simulink model "StarshipSystemModel"  (R2025b)
settings: Solver=VariableStepAuto  StartTime=0.0  StopTime=10.0  RelTol=1e-3
model workspace (MAT data in the model file):
  ActiveGNCMode : Simulink.Bus (value not decoded)
  AerodynamicControlCommand : Simulink.Bus (value not decoded)
  AerodynamicLoad : Simulink.Bus (value not decoded)
  AggregatedStream : Simulink.Bus (value not decoded)
  AllocatedEffectorDemand : Simulink.Bus (value not decoded)
  AttitudeControlDemand : Simulink.Bus (value not decoded)
  AttitudeGuidanceCommand : Simulink.Bus (value not decoded)
  AttitudeRateState : Simulink.Bus (value not decoded)
  AutogenousPressurantGas : Simulink.ConnectionBus (value not decoded)
  CandidateFaultIndication : Simulink.Bus (value not decoded)
  CombustionGasFeed : Simulink.ConnectionBus (value not decoded)
  CommandPathHealth : Simulink.Bus (value not decoded)
  ControlMode : Simulink.ValueType (value not decoded)
  DownlinkSignal : Simulink.Bus (value not decoded)
  ElectricalPower : Simulink.ConnectionBus (value not decoded)
  EngineTelemetry : Simulink.Bus (value not decoded)
  ExecutionContext : Simulink.Bus (value not decoded)
  FaultDiagnosisResult : Simulink.Bus (value not decoded)
  GNCDataContext : Simulink.Bus (value not decoded)
  GNCHealthState : Simulink.Bus (value not decoded)
  GNCStateEstimate : Simulink.Bus (value not decoded)
  GimbalAngle : Simulink.ValueType (value not decoded)
  GimbalMotion : Simulink.ConnectionBus (value not decoded)
  GroundCheckoutLink : Simulink.Bus (value not decoded)
  GroundPressurantSupply : Simulink.ConnectionBus (value not decoded)
  GuidanceConstraints : Simulink.Bus (value not decoded)
  GuidanceMode : Simulink.ValueType (value not decoded)
  LinkHealth : Simulink.Bus (value not decoded)
  LiquidPropellantFeed : Simulink.ConnectionBus (value not decoded)
  MechanicalMotion : Simulink.ConnectionBus (value not decoded)
  MechanismPosition : Simulink.Bus (value not decoded)
  ModeTransitionContext : Simulink.Bus (value not decoded)
  NavigationAidingData : Simulink.Bus (value not decoded)
  NavigationEstimate : Simulink.Bus (value not decoded)
  NavigationHealthStatus : Simulink.Bus (value not decoded)
  NavigationMeasurementSet : Simulink.Bus (value not decoded)
  PercentThrottle : Simulink.ValueType (value not decoded)
  PneumaticActuationGas : Simulink.ConnectionBus (value not decoded)
  PowerConversionStatus : Simulink.Bus (value not decoded)
  PowerDistributionStatus : Simulink.Bus (value not decoded)
  PowerHealthStatus : Simulink.Bus (value not decoded)
  PowerManagementCommand : Simulink.Bus (value not decoded)
  PowerStorageStatus : Simulink.Bus (value not decoded)
  ProtectedThermalState : Simulink.Bus (value not decoded)
  ProtectionIsolationStatus : Simulink.Bus (value not decoded)
  PurgeGasSupply : Simulink.ConnectionBus (value not decoded)
  RCSPulseCommand : Simulink.Bus (value not decoded)
  RCSTelemetry : Simulink.Bus (value not decoded)
  RFFeed : Simulink.ConnectionBus (value not decoded)
  RecoveryMechanismCommand : Simulink.Bus (value not decoded)
  RollThrottleBias : Simulink.ValueType (value not decoded)
  SafetyOverride : Simulink.ValueType (value not decoded)
  SafetyStateStatus : Simulink.Bus (value not decoded)
  ShapedControlDemand : Simulink.Bus (value not decoded)
  SpinStartIgniterGas : Simulink.ConnectionBus (value not decoded)
  StageMechanicalBoundary : Simulink.ConnectionBus (value not decoded)
  StructuralLoad : Simulink.ConnectionBus (value not decoded)
  StructureHealthStatus : Simulink.Bus (value not decoded)
  SubsystemHealthEvidence : Simulink.Bus (value not decoded)
  SubsystemStatusTelemetry : Simulink.Bus (value not decoded)
  TankTelemetry : Simulink.Bus (value not decoded)
  ThermalMonitoringCommand : Simulink.Bus (value not decoded)
  ThermalNetwork : Simulink.ConnectionBus (value not decoded)
  ThrustLoad : Simulink.ConnectionBus (value not decoded)
  TrajectoryGuidanceCommand : Simulink.Bus (value not decoded)
  TrajectoryReference : Simulink.Bus (value not decoded)
  TranslationalControlDemand : Simulink.Bus (value not decoded)
  TranslationalState : Simulink.Bus (value not decoded)
  UplinkSignal : Simulink.Bus (value not decoded)
  ValidatedControlDemand : Simulink.Bus (value not decoded)
  ValveCommand : Simulink.ValueType (value not decoded)
  VehicleStructureState : Simulink.Bus (value not decoded)
  VerifiedCommand : Simulink.Bus (value not decoded)
  VideoStream : Simulink.Bus (value not decoded)
undefined symbols (not defined in the file): ACR, ACT, ASM, ATM, BCR, BDQ, BDR, BDX, BEC, BFC, BHV, BIP, BLM, BNZ, BPI, BPR, BPV, BRX, BSM, BTA, BTP, BVC, BVE, BVV, CAA, CAM, CAS, CAT, CLM, COM, CRS, CTL, CTR, DAQ, ESC, EXT, FCR, FDB, FDE, FEX, FHI, FHM, FIC, FIS, FMG, FSC, GAP, GCM, GMD, GNC, GND, GPH, GTR, HDN, HIA, HSI, IF, INT, LOC, NAI ... (+45)
(part 7 of 8)

== system StarshipSystemModel/Starship/Power & Electrical Energy/Power Conversion & Conditioning/Inverter // Conversion Function ==
  IF-BES-INV-01 : PMIOPort  Side=Left  ConnectionType=Bus: ElectricalPower
  IF-INV-PCR-01 : PMIOPort  Port=2  Side=Right  ConnectionType=Bus: ElectricalPower

== system StarshipSystemModel/Starship/Power & Electrical Energy/Power Conversion & Conditioning/Power Conditioning // Regulation ==
  IF-INV-PCR-01 : PMIOPort  Side=Left  ConnectionType=Bus: ElectricalPower
  IF-PCR-HDN-01 : PMIOPort  Port=2  Side=Right  ConnectionType=Bus: ElectricalPower

== system StarshipSystemModel/Starship/Power & Electrical Energy/Power Management & Monitoring/Power Management Coordinator ==
  Bus Element In1 : Inport  PortName=IF-PSM-PMC-01
  Bus Element Out1 : Outport  PortName=IF-PMC-BIP-01
  Bus Element Out2 : Outport  Port=2  PortName=IF-PMC-HSI-01
  Bus Element Out3 : Outport  Port=3  PortName=IF-PMM-SAF-01

== system StarshipSystemModel/Starship/Power & Electrical Energy/Power Management & Monitoring/Power State Monitor ==
  Bus Element In3 : Inport  PortName=IF-HDN-PSM-01
  Bus Element In2 : Inport  Port=2  PortName=IF-PCM-PSM-01
  Bus Element In1 : Inport  Port=3  PortName=IF-BSM-PSM-01
  Bus Element Out1 : Outport  PortName=IF-PSM-PMC-01

== system StarshipSystemModel/Starship/Power & Electrical Energy/Power Management & Monitoring/Protection // Isolation Status ==
  Bus Element In1 : Inport  PortName=IF-BIP-PIS-01
  Bus Element In2 : Inport  Port=2  PortName=IF-HSI-PIS-01
  Bus Element In3 : Inport  Port=3  PortName=IF-BPI-PIS-01

== system StarshipSystemModel/Starship/Propellent system/Booster propellant System/Booster propellant tanks ==
  Anti-slosh baffles : Subsystem
      settings: PortSchema="{\"entries\":[{\"content\":{\"headerSize\":26,\"margin\":15,\"minimumSpacing\":25,\"sides\":[{\"content\":{},\"type\":\"ConnectorPlacement.EquallySpacedRectSide\",\"uuid\":\"fbe4f8e6-132c-4a0c-8c4c-52d0209da778\"},{\"content\":{\"side\":\"RIGHT\"},\"type\":\"ConnectorPlacement.EquallySpacedRectSide\",\"uuid\":\"bbe80fa3-b8e3-44c5-9574-5758a55378fd\"},{\"content\":{\"side\":\"TOP\"},\"type\":\"ConnectorPlacement.EquallySpacedRectSide\",\"uuid\":\"410005e2-e10b-4d3e-a617-d51b1ea5de7e\"}]},\"type\":\"ConnectorPlacement.EquallySpacedConnector\",\"uuid\":\"b66a347a-e5b4-46b1-8a3f-28cf70f30a27\"}],\"packageUris\":[\"http://schema.mathworks.com/mf0/Connector/R2020b\"],\"version\":\"1.0\"}"
  CH4 main tank : Subsystem
      settings: PortSchema="{\"entries\":[{\"content\":{\"headerSize\":26,\"margin\":15,\"minimumSpacing\":25,\"sides\":[{\"content\":{\"connectorIds\":[\"LConn1\",\"LConn2\"]},\"type\":\"ConnectorPlacement.EquallySpacedRectSide\",\"uuid\":\"fbe4f8e6-132c-4a0c-8c4c-52d0209da778\"},{\"content\":{\"connectorIds\":[\"RConn1\",\"RConn2\"],\"side\":\"RIGHT\"},\"type\":\"ConnectorPlacement.EquallySpacedRectSide\",\"uuid\":\"bbe80fa3-b8e3-44c5-9574-5758a55378fd\"},{\"content\":{\"side\":\"TOP\"},\"type\":\"ConnectorPlacement.EquallySpacedRectSide\",\"uuid\":\"410005e2-e10b-4d3e-a617-d51b1ea5de7e\"}]},\"type\":\"ConnectorPlacement.EquallySpacedConnector\",\"uuid\":\"b66a347a-e5b4-46b1-8a3f-28cf70f30a27\"}],\"packageUris\":[\"http://schema.mathworks.com/mf0/Connector/R2020b\"],\"version\":\"1.0\"}"
  CH4 transfer tube (downcomer) : Subsystem
      settings: PortSchema="{\"entries\":[{\"content\":{\"headerSize\":26,\"margin\":15,\"minimumSpacing\":25,\"sides\":[{\"content\":{},\"type\":\"ConnectorPlacement.EquallySpacedRectSide\",\"uuid\":\"fbe4f8e6-132c-4a0c-8c4c-52d0209da778\"},{\"content\":{\"side\":\"RIGHT\"},\"type\":\"ConnectorPlacement.EquallySpacedRectSide\",\"uuid\":\"bbe80fa3-b8e3-44c5-9574-5758a55378fd\"},{\"content\":{\"side\":\"TOP\"},\"type\":\"ConnectorPlacement.EquallySpacedRectSide\",\"uuid\":\"410005e2-e10b-4d3e-a617-d51b1ea5de7e\"}]},\"type\":\"ConnectorPlacement.EquallySpacedConnector\",\"uuid\":\"b66a347a-e5b4-46b1-8a3f-28cf70f30a27\"}],\"packageUris\":[\"http://schema.mathworks.com/mf0/Connector/R2020b\"],\"version\":\"1.0\"}"
  Common dome : Subsystem
      settings: PortSchema="{\"entries\":[{\"content\":{\"headerSize\":26,\"margin\":15,\"minimumSpacing\":25,\"sides\":[{\"content\":{},\"type\":\"ConnectorPlacement.EquallySpacedRectSide\",\"uuid\":\"fbe4f8e6-132c-4a0c-8c4c-52d0209da778\"},{\"content\":{\"side\":\"RIGHT\"},\"type\":\"ConnectorPlacement.EquallySpacedRectSide\",\"uuid\":\"bbe80fa3-b8e3-44c5-9574-5758a55378fd\"},{\"content\":{\"side\":\"TOP\"},\"type\":\"ConnectorPlacement.EquallySpacedRectSide\",\"uuid\":\"410005e2-e10b-4d3e-a617-d51b1ea5de7e\"}]},\"type\":\"ConnectorPlacement.EquallySpacedConnector\",\"uuid\":\"b66a347a-e5b4-46b1-8a3f-28cf70f30a27\"}],\"packageUris\":[\"http://schema.mathworks.com/mf0/Connector/R2020b\"],\"version\":\"1.0\"}"
  LOX landing tank : Subsystem
      settings: PortSchema="{\"entries\":[{\"content\":{\"headerSize\":26,\"margin\":15,\"minimumSpacing\":25,\"sides\":[{\"content\":{},\"type\":\"ConnectorPlacement.EquallySpacedRectSide\",\"uuid\":\"fbe4f8e6-132c-4a0c-8c4c-52d0209da778\"},{\"content\":{\"connectorIds\":[\"RConn1\"],\"side\":\"RIGHT\"},\"type\":\"ConnectorPlacement.EquallySpacedRectSide\",\"uuid\":\"bbe80fa3-b8e3-44c5-9574-5758a55378fd\"},{\"content\":{\"side\":\"TOP\"},\"type\":\"ConnectorPlacement.EquallySpacedRectSide\",\"uuid\":\"410005e2-e10b-4d3e-a617-d51b1ea5de7e\"}]},\"type\":\"ConnectorPlacement.EquallySpacedConnector\",\"uuid\":\"b66a347a-e5b4-46b1-8a3f-28cf70f30a27\"}],\"packageUris\":[\"http://schema.mathworks.com/mf0/Connector/R2020b\"],\"version\":\"1.0\"}"
  LOX main tank : Subsystem
      settings: PortSchema="{\"entries\":[{\"content\":{\"headerSize\":26,\"margin\":15,\"minimumSpacing\":25,\"sides\":[{\"content\":{\"connectorIds\":[\"LConn2\",\"LConn3\"]},\"type\":\"ConnectorPlacement.EquallySpacedRectSide\",\"uuid\":\"fbe4f8e6-132c-4a0c-8c4c-52d0209da778\"},{\"content\":{\"connectorIds\":[\"LConn1\",\"RConn1\",\"RConn2\"],\"side\":\"RIGHT\"},\"type\":\"ConnectorPlacement.EquallySpacedRectSide\",\"uuid\":\"bbe80fa3-b8e3-44c5-9574-5758a55378fd\"},{\"content\":{\"side\":\"TOP\"},\"type\":\"ConnectorPlacement.EquallySpacedRectSide\",\"uuid\":\"410005e2-e10b-4d3e-a617-d51b1ea5de7e\"}]},\"type\":\"ConnectorPlacement.EquallySpacedConnector\",\"uuid\":\"b66a347a-e5b4-46b1-8a3f-28cf70f30a27\"}],\"packageUris\":[\"http://schema.mathworks.com/mf0/Connector/R2020b\"],\"version\":\"1.0\"}"
  IF-BOT-BPV-01 : PMIOPort  Side=Right
  IF-BFT-BPV-01 : PMIOPort  Port=2  Side=Right  ConnectionType=Bus: LiquidPropellantFeed
  IF-BFT-BVV-01 : PMIOPort  Port=3  Side=Right  ConnectionType=Bus: AutogenousPressurantGas
  IF-BOT-BVV-01 : PMIOPort  Port=4  Side=Right  ConnectionType=Bus: AutogenousPressurantGas
  IF-BLT-BHV-01 : PMIOPort  Port=5  Side=Right  ConnectionType=Bus: LiquidPropellantFeed
  IF-BOT-PRS-01 : PMIOPort  Port=6  Side=Left  ConnectionType=Bus: StructuralLoad
  IF-BCQ-BFT-01 : PMIOPort  Port=7  Side=Left  ConnectionType=Bus: LiquidPropellantFeed
  IF-BPR-BOT-01 : PMIOPort  Port=8  Side=Left  ConnectionType=Bus: AutogenousPressurantGas
  IF-BLQ-BOT-01 : PMIOPort  Port=9  Side=Left  ConnectionType=Bus: LiquidPropellantFeed
  IF-BPR-BFT-01 : PMIOPort  Port=10  Side=Left  ConnectionType=Bus: AutogenousPressurantGas
  connections:
  IF-BPR-BOT-01/RConn1 -- LOX main tank/LConn2
  IF-BPR-BFT-01/RConn1 -- CH4 main tank/LConn2
  IF-BLQ-BOT-01/RConn1 -- LOX main tank/LConn3
  IF-BCQ-BFT-01/RConn1 -- CH4 main tank/LConn1
  CH4 main tank/RConn1 -- IF-BFT-BPV-01/RConn1
  LOX landing tank/RConn1 -- IF-BLT-BHV-01/RConn1
  LOX main tank/RConn1 -- IF-BOT-BPV-01/RConn1
  LOX main tank/RConn2 -- IF-BOT-BVV-01/RConn1
  CH4 main tank/RConn2 -- IF-BFT-BVV-01/RConn1
  IF-BOT-PRS-01/RConn1 -- LOX main tank/LConn1

== system StarshipSystemModel/Starship/Propellent system/Booster propellant System/Feed & distribution ==
  Bus Element In1 : Inport  PortName=IF-GNC-BFC-01
  Distribution manifold : Subsystem
      settings: PortSchema="{\"entries\":[{\"content\":{\"headerSize\":26,\"margin\":15,\"minimumSpacing\":25,\"sides\":[{\"content\":{\"connectorIds\":[\"LConn1\",\"LConn2\"]},\"type\":\"ConnectorPlacement.EquallySpacedRectSide\",\"uuid\":\"fbe4f8e6-132c-4a0c-8c4c-52d0209da778\"},{\"content\":{\"connectorIds\":[\"RConn1\"],\"side\":\"RIGHT\"},\"type\":\"ConnectorPlacement.EquallySpacedRectSide\",\"uuid\":\"bbe80fa3-b8e3-44c5-9574-5758a55378fd\"},{\"content\":{\"side\":\"TOP\"},\"type\":\"ConnectorPlacement.EquallySpacedRectSide\",\"uuid\":\"410005e2-e10b-4d3e-a617-d51b1ea5de7e\"}]},\"type\":\"ConnectorPlacement.EquallySpacedConnector\",\"uuid\":\"b66a347a-e5b4-46b1-8a3f-28cf70f30a27\"}],\"packageUris\":[\"http://schema.mathworks.com/mf0/Connector/R2020b\"],\"version\":\"1.0\"}"
  Feed controller : Subsystem
      settings: PortSchema="{\"entries\":[{\"content\":{\"headerSize\":26,\"margin\":15,\"minimumSpacing\":25,\"sides\":[{\"content\":{\"connectorIds\":[\"In1\",\"LConn1\"]},\"type\":\"ConnectorPlacement.EquallySpacedRectSide\",\"uuid\":\"fbe4f8e6-132c-4a0c-8c4c-52d0209da778\"},{\"content\":{\"connectorIds\":[\"Out1\",\"Out2\"],\"side\":\"RIGHT\"},\"type\":\"ConnectorPlacement.EquallySpacedRectSide\",\"uuid\":\"bbe80fa3-b8e3-44c5-9574-5758a55378fd\"},{\"content\":{\"side\":\"TOP\"},\"type\":\"ConnectorPlacement.EquallySpacedRectSide\",\"uuid\":\"410005e2-e10b-4d3e-a617-d51b1ea5de7e\"}]},\"type\":\"ConnectorPlacement.EquallySpacedConnector\",\"uuid\":\"b66a347a-e5b4-46b1-8a3f-28cf70f30a27\"}],\"packageUris\":[\"http://schema.mathworks.com/mf0/Connector/R2020b\"],\"version\":\"1.0\"}"
  Header tank switchover valve : Subsystem
      settings: PortSchema="{\"entries\":[{\"content\":{\"headerSize\":26,\"margin\":15,\"minimumSpacing\":25,\"sides\":[{\"content\":{\"connectorIds\":[\"LConn1\",\"In1\",\"LConn2\"]},\"type\":\"ConnectorPlacement.EquallySpacedRectSide\",\"uuid\":\"fbe4f8e6-132c-4a0c-8c4c-52d0209da778\"},{\"content\":{\"connectorIds\":[\"RConn1\"],\"side\":\"RIGHT\"},\"type\":\"ConnectorPlacement.EquallySpacedRectSide\",\"uuid\":\"bbe80fa3-b8e3-44c5-9574-5758a55378fd\"},{\"content\":{\"side\":\"TOP\"},\"type\":\"ConnectorPlacement.EquallySpacedRectSide\",\"uuid\":\"410005e2-e10b-4d3e-a617-d51b1ea5de7e\"}]},\"type\":\"ConnectorPlacement.EquallySpacedConnector\",\"uuid\":\"b66a347a-e5b4-46b1-8a3f-28cf70f30a27\"}],\"packageUris\":[\"http://schema.mathworks.com/mf0/Connector/R2020b\"],\"version\":\"1.0\"}"
  Main tank outlet valve (prevalve) : Subsystem
      settings: PortSchema="{\"entries\":[{\"content\":{\"headerSize\":26,\"margin\":15,\"minimumSpacing\":25,\"sides\":[{\"content\":{\"connectorIds\":[\"LConn1\",\"LConn2\",\"In1\",\"LConn3\"]},\"type\":\"ConnectorPlacement.EquallySpacedRectSide\",\"uuid\":\"fbe4f8e6-132c-4a0c-8c4c-52d0209da778\"},{\"content\":{\"connectorIds\":[\"RConn1\"],\"side\":\"RIGHT\"},\"type\":\"ConnectorPlacement.EquallySpacedRectSide\",\"uuid\":\"bbe80fa3-b8e3-44c5-9574-5758a55378fd\"},{\"content\":{\"side\":\"TOP\"},\"type\":\"ConnectorPlacement.EquallySpacedRectSide\",\"uuid\":\"410005e2-e10b-4d3e-a617-d51b1ea5de7e\"}]},\"type\":\"ConnectorPlacement.EquallySpacedConnector\",\"uuid\":\"b66a347a-e5b4-46b1-8a3f-28cf70f30a27\"}],\"packageUris\":[\"http://schema.mathworks.com/mf0/Connector/R2020b\"],\"version\":\"1.0\"}"
  IF-BDM-BTP-01 : PMIOPort  Side=Right  ConnectionType=Bus: LiquidPropellantFeed
  IF-BOT-BPV-01 : PMIOPort  Port=2  Side=Left  ConnectionType=Bus: LiquidPropellantFeed
  IF-BLT-BHV-01 : PMIOPort  Port=3  Side=Left  ConnectionType=Bus: LiquidPropellantFeed
  IF-BNG-BPV-01 : PMIOPort  Port=4  Side=Left  ConnectionType=Bus: PneumaticActuationGas
  IF-BNG-BHV-01 : PMIOPort  Port=5  Side=Left  ConnectionType=Bus: PneumaticActuationGas
  IF-BFT-BPV-01 : PMIOPort  Port=6  Side=Left  ConnectionType=Bus: LiquidPropellantFeed
  IF-PWR-BFC-01 : PMIOPort  Port=7  Side=Left  ConnectionType=Bus: ElectricalPower
  wires:
  Bus Element In1/1 -> Feed controller/1(IF-GNC-BFC-01)
  Feed controller/2(IF-BFC-BHV-01) -> Header tank switchover valve/1(IF-BFC-BHV-01)
  Feed controller/1(IF-BFC-BPV-01) -> Main tank outlet valve (prevalve)/1(IF-BFC-BPV-01)
  connections:
  IF-BLT-BHV-01/RConn1 -- Header tank switchover valve/LConn1
  IF-BFT-BPV-01/RConn1 -- Main tank outlet valve (prevalve)/LConn2
  Header tank switchover valve/RConn1 -- Distribution manifold/LConn1
  IF-BNG-BHV-01/RConn1 -- Header tank switchover valve/LConn2
  IF-BOT-BPV-01/RConn1 -- Main tank outlet valve (prevalve)/LConn1
  IF-BNG-BPV-01/RConn1 -- Main tank outlet valve (prevalve)/LConn3
  Main tank outlet valve (prevalve)/RConn1 -- Distribution manifold/LConn2
  Distribution manifold/RConn1 -- IF-BDM-BTP-01/RConn1
  IF-PWR-BFC-01/RConn1 -- Feed controller/LConn1

== system StarshipSystemModel/Starship/Propellent system/Booster propellant System/Ground propellant interface ==
  CH4 quick-disconnect panel : Subsystem
      settings: PortSchema="{\"entries\":[{\"content\":{\"headerSize\":26,\"margin\":15,\"minimumSpacing\":25,\"sides\":[{\"content\":{\"connectorIds\":[\"LConn1\"]},\"type\":\"ConnectorPlacement.EquallySpacedRectSide\",\"uuid\":\"fbe4f8e6-132c-4a0c-8c4c-52d0209da778\"},{\"content\":{\"connectorIds\":[\"RConn1\"],\"side\":\"RIGHT\"},\"type\":\"ConnectorPlacement.EquallySpacedRectSide\",\"uuid\":\"bbe80fa3-b8e3-44c5-9574-5758a55378fd\"},{\"content\":{\"side\":\"TOP\"},\"type\":\"ConnectorPlacement.EquallySpacedRectSide\",\"uuid\":\"410005e2-e10b-4d3e-a617-d51b1ea5de7e\"}]},\"type\":\"ConnectorPlacement.EquallySpacedConnector\",\"uuid\":\"b66a347a-e5b4-46b1-8a3f-28cf70f30a27\"}],\"packageUris\":[\"http://schema.mathworks.com/mf0/Connector/R2020b\"],\"version\":\"1.0\"}"
  LOX quick-disconnect panel : Subsystem
      settings: PortSchema="{\"entries\":[{\"content\":{\"headerSize\":26,\"margin\":15,\"minimumSpacing\":25,\"sides\":[{\"content\":{\"connectorIds\":[\"LConn1\"]},\"type\":\"ConnectorPlacement.EquallySpacedRectSide\",\"uuid\":\"fbe4f8e6-132c-4a0c-8c4c-52d0209da778\"},{\"content\":{\"connectorIds\":[\"RConn1\"],\"side\":\"RIGHT\"},\"type\":\"ConnectorPlacement.EquallySpacedRectSide\",\"uuid\":\"bbe80fa3-b8e3-44c5-9574-5758a55378fd\"},{\"content\":{\"side\":\"TOP\"},\"type\":\"ConnectorPlacement.EquallySpacedRectSide\",\"uuid\":\"410005e2-e10b-4d3e-a617-d51b1ea5de7e\"}]},\"type\":\"ConnectorPlacement.EquallySpacedConnector\",\"uuid\":\"b66a347a-e5b4-46b1-8a3f-28cf70f30a27\"}],\"packageUris\":[\"http://schema.mathworks.com/mf0/Connector/R2020b\"],\"version\":\"1.0\"}"
  Purge/pressurant ground QD : Subsystem
      settings: PortSchema="{\"entries\":[{\"content\":{\"headerSize\":26,\"margin\":15,\"minimumSpacing\":25,\"sides\":[{\"content\":{\"connectorIds\":[\"LConn1\"]},\"type\":\"ConnectorPlacement.EquallySpacedRectSide\",\"uuid\":\"fbe4f8e6-132c-4a0c-8c4c-52d0209da778\"},{\"content\":{\"connectorIds\":[\"RConn1\",\"RConn2\",\"RConn3\"],\"side\":\"RIGHT\"},\"type\":\"ConnectorPlacement.EquallySpacedRectSide\",\"uuid\":\"bbe80fa3-b8e3-44c5-9574-5758a55378fd\"},{\"content\":{\"side\":\"TOP\"},\"type\":\"ConnectorPlacement.EquallySpacedRectSide\",\"uuid\":\"410005e2-e10b-4d3e-a617-d51b1ea5de7e\"}]},\"type\":\"ConnectorPlacement.EquallySpacedConnector\",\"uuid\":\"b66a347a-e5b4-46b1-8a3f-28cf70f30a27\"}],\"packageUris\":[\"http://schema.mathworks.com/mf0/Connector/R2020b\"],\"version\":\"1.0\"}"
  "IF-GND-BLQ-01\t" : PMIOPort  Side=Left
  "IF-GND-BCQ-01\t" : PMIOPort  Port=2  Side=Left
  IF-GND-BPQ-01 : PMIOPort  Port=3  Side=Left  ConnectionType=Bus: GroundPressurantSupply
  IF-BCQ-BFT-01 : PMIOPort  Port=4  Side=Right  ConnectionType=Bus: LiquidPropellantFeed
  IF-BPQ-BSG-01 : PMIOPort  Port=5  Side=Right  ConnectionType=Bus: GroundPressurantSupply
  IF-BPQ-BNG-01 : PMIOPort  Port=6  Side=Right  ConnectionType=Bus: GroundPressurantSupply
  IF-BPQ-BPR-01 : PMIOPort  Port=7  Side=Right  ConnectionType=Bus: GroundPressurantSupply
  IF-BLQ-BOT-01 : PMIOPort  Port=8  Side=Right  ConnectionType=Bus: LiquidPropellantFeed
  connections:
  Purge/pressurant ground QD/RConn1 -- IF-BPQ-BSG-01/RConn1
  IF-GND-BPQ-01/RConn1 -- Purge/pressurant ground QD/LConn1
  "IF-GND-BLQ-01\t"/RConn1 -- LOX quick-disconnect panel/LConn1
  Purge/pressurant ground QD/RConn3 -- IF-BPQ-BNG-01/RConn1
  CH4 quick-disconnect panel/RConn1 -- IF-BCQ-BFT-01/RConn1
  "IF-GND-BCQ-01\t"/RConn1 -- CH4 quick-disconnect panel/LConn1
  Purge/pressurant ground QD/RConn2 -- IF-BPQ-BPR-01/RConn1
  LOX quick-disconnect panel/RConn1 -- IF-BLQ-BOT-01/RConn1

== system StarshipSystemModel/Starship/Propellent system/Booster propellant System/Pressurization, purge & venting ==
  Bus Element In1 : Inport  PortName=IF-GNC-BPR-01
  Autogenous pressurization regulator : Subsystem
      settings: PortSchema="{\"entries\":[{\"content\":{\"headerSize\":26,\"margin\":15,\"minimumSpacing\":25,\"sides\":[{\"content\":{\"connectorIds\":[\"LConn1\",\"LConn2\",\"In1\",\"LConn3\"]},\"type\":\"ConnectorPlacement.EquallySpacedRectSide\",\"uuid\":\"fbe4f8e6-132c-4a0c-8c4c-52d0209da778\"},{\"content\":{\"connectorIds\":[\"Out1\",\"Out2\",\"RConn1\",\"RConn2\",\"Out3\"],\"side\":\"RIGHT\"},\"type\":\"ConnectorPlacement.EquallySpacedRectSide\",\"uuid\":\"bbe80fa3-b8e3-44c5-9574-5758a55378fd\"},{\"content\":{\"side\":\"TOP\"},\"type\":\"ConnectorPlacement.EquallySpacedRectSide\",\"uuid\":\"410005e2-e10b-4d3e-a617-d51b1ea5de7e\"}]},\"type\":\"ConnectorPlacement.EquallySpacedConnector\",\"uuid\":\"b66a347a-e5b4-46b1-8a3f-28cf70f30a27\"}],\"packageUris\":[\"http://schema.mathworks.com/mf0/Connector/R2020b\"],\"version\":\"1.0\"}"
  Pneumatic actuation gas COPVs : Subsystem
      settings: PortSchema="{\"entries\":[{\"content\":{\"headerSize\":26,\"margin\":15,\"minimumSpacing\":25,\"sides\":[{\"content\":{\"connectorIds\":[\"LConn1\"]},\"type\":\"ConnectorPlacement.EquallySpacedRectSide\",\"uuid\":\"fbe4f8e6-132c-4a0c-8c4c-52d0209da778\"},{\"content\":{\"connectorIds\":[\"RConn1\",\"RConn2\",\"RConn3\",\"RConn4\"],\"side\":\"RIGHT\"},\"type\":\"ConnectorPlacement.EquallySpacedRectSide\",\"uuid\":\"bbe80fa3-b8e3-44c5-9574-5758a55378fd\"},{\"content\":{\"side\":\"TOP\"},\"type\":\"ConnectorPlacement.EquallySpacedRectSide\",\"uuid\":\"410005e2-e10b-4d3e-a617-d51b1ea5de7e\"}]},\"type\":\"ConnectorPlacement.EquallySpacedConnector\",\"uuid\":\"b66a347a-e5b4-46b1-8a3f-28cf70f30a27\"}],\"packageUris\":[\"http://schema.mathworks.com/mf0/Connector/R2020b\"],\"version\":\"1.0\"}"
  Spin-start & igniter gas COPVs : Subsystem
      settings: PortSchema="{\"entries\":[{\"content\":{\"headerSize\":26,\"margin\":15,\"minimumSpacing\":25,\"sides\":[{\"content\":{\"connectorIds\":[\"LConn1\"]},\"type\":\"ConnectorPlacement.EquallySpacedRectSide\",\"uuid\":\"fbe4f8e6-132c-4a0c-8c4c-52d0209da778\"},{\"content\":{\"connectorIds\":[\"RConn1\"],\"side\":\"RIGHT\"},\"type\":\"ConnectorPlacement.EquallySpacedRectSide\",\"uuid\":\"bbe80fa3-b8e3-44c5-9574-5758a55378fd\"},{\"content\":{\"side\":\"TOP\"},\"type\":\"ConnectorPlacement.EquallySpacedRectSide\",\"uuid\":\"410005e2-e10b-4d3e-a617-d51b1ea5de7e\"}]},\"type\":\"ConnectorPlacement.EquallySpacedConnector\",\"uuid\":\"b66a347a-e5b4-46b1-8a3f-28cf70f30a27\"}],\"packageUris\":[\"http://schema.mathworks.com/mf0/Connector/R2020b\"],\"version\":\"1.0\"}"
  Vent & relief valves : Subsystem
      settings: PortSchema="{\"entries\":[{\"content\":{\"headerSize\":26,\"margin\":15,\"minimumSpacing\":25,\"sides\":[{\"content\":{\"connectorIds\":[\"In1\",\"LConn1\",\"LConn2\",\"LConn3\"]},\"type\":\"ConnectorPlacement.EquallySpacedRectSide\",\"uuid\":\"fbe4f8e6-132c-4a0c-8c4c-52d0209da778\"},{\"content\":{\"side\":\"RIGHT\"},\"type\":\"ConnectorPlacement.EquallySpacedRectSide\",\"uuid\":\"bbe80fa3-b8e3-44c5-9574-5758a55378fd\"},{\"content\":{\"side\":\"TOP\"},\"type\":\"ConnectorPlacement.EquallySpacedRectSide\",\"uuid\":\"410005e2-e10b-4d3e-a617-d51b1ea5de7e\"}]},\"type\":\"ConnectorPlacement.EquallySpacedConnector\",\"uuid\":\"b66a347a-e5b4-46b1-8a3f-28cf70f30a27\"}],\"packageUris\":[\"http://schema.mathworks.com/mf0/Connector/R2020b\"],\"version\":\"1.0\"}"
  IF-BSG-BIG-01 : PMIOPort  Side=Right  ConnectionType=Bus: SpinStartIgniterGas
  IF-BPR-BFT-01 : PMIOPort  Port=2  Side=Right  ConnectionType=Bus: AutogenousPressurantGas
  IF-BNG-BPV-01 : PMIOPort  Port=3  Side=Right  ConnectionType=Bus: PneumaticActuationGas
  IF-BNG-BHV-01 : PMIOPort  Port=4  Side=Right  ConnectionType=Bus: PneumaticActuationGas
  IF-BPR-BOT-01 : PMIOPort  Port=5  Side=Right  ConnectionType=Bus: AutogenousPressurantGas
  IF-BNG-BVC-01 : PMIOPort  Port=6  Side=Right  ConnectionType=Bus: PneumaticActuationGas
  IF-BPQ-BPR-01 : PMIOPort  Port=7  Side=Left  ConnectionType=Bus: GroundPressurantSupply
  IF-BPQ-BNG-01 : PMIOPort  Port=8  Side=Left  ConnectionType=Bus: GroundPressurantSupply
  IF-BPQ-BSG-01 : PMIOPort  Port=9  Side=Left  ConnectionType=Bus: GroundPressurantSupply
  IF-BTP-BPR-01 : PMIOPort  Port=10  Side=Left  ConnectionType=Bus: AutogenousPressurantGas
  IF-BOT-BVV-01 : PMIOPort  Port=11  Side=Left  ConnectionType=Bus: AutogenousPressurantGas
  IF-BFT-BVV-01 : PMIOPort  Port=12  Side=Left  ConnectionType=Bus: AutogenousPressurantGas
  IF-PWR-BPR-01 : PMIOPort  Port=13  Side=Left  ConnectionType=Bus: ElectricalPower
  Bus Element Out2 : Outport  PortName=IF-BPR-BTA-01
  Bus Element Out1 : Outport  Port=2  PortName=IF-BPR-SAF-01
  wires:
  Autogenous pressurization regulator/1(IF-BPR-SAF-01) -> Bus Element Out1/1
  Bus Element In1/1 -> Autogenous pressurization regulator/1(IF-GNC-BPR-01)
  Autogenous pressurization regulator/2(IF-BPR-COM-01) -> Bus Element Out2/1
  Autogenous pressurization regulator/3(IF-BPR-BVV-01) -> Vent & relief valves/1(IF-BPR-BVV-01)
  connections:
  IF-BPQ-BSG-01/RConn1 -- Spin-start & igniter gas COPVs/LConn1
  IF-BPQ-BNG-01/RConn1 -- Pneumatic actuation gas COPVs/LConn1
  IF-BPQ-BPR-01/RConn1 -- Autogenous pressurization regulator/LConn1
  Autogenous pressurization regulator/RConn2 -- IF-BPR-BFT-01/RConn1
  Autogenous pressurization regulator/RConn1 -- IF-BPR-BOT-01/RConn1
  IF-BTP-BPR-01/RConn1 -- Autogenous pressurization regulator/LConn2
  IF-BOT-BVV-01/RConn1 -- Vent & relief valves/LConn2
  IF-BFT-BVV-01/RConn1 -- Vent & relief valves/LConn1
  Pneumatic actuation gas COPVs/RConn4 -- Vent & relief valves/LConn3
  Pneumatic actuation gas COPVs/RConn1 -- IF-BNG-BHV-01/RConn1
  Pneumatic actuation gas COPVs/RConn2 -- IF-BNG-BPV-01/RConn1
  Pneumatic actuation gas COPVs/RConn3 -- IF-BNG-BVC-01/RConn1
  Spin-start & igniter gas COPVs/RConn1 -- IF-BSG-BIG-01/RConn1
  IF-PWR-BPR-01/RConn1 -- Autogenous pressurization regulator/LConn3

== system StarshipSystemModel/Starship/Propellent system/Ship propellant System/Feed & distribution ==
  Bus Element In1 : Inport  PortName=IF-GNC-SFC-01
  Distribution manifold : Subsystem
      settings: PortSchema="{\"entries\":[{\"content\":{\"headerSize\":26,\"margin\":15,\"minimumSpacing\":25,\"sides\":[{\"content\":{\"connectorIds\":[\"LConn1\",\"LConn2\"]},\"type\":\"ConnectorPlacement.EquallySpacedRectSide\",\"uuid\":\"fbe4f8e6-132c-4a0c-8c4c-52d0209da778\"},{\"content\":{\"connectorIds\":[\"RConn1\"],\"side\":\"RIGHT\"},\"type\":\"ConnectorPlacement.EquallySpacedRectSide\",\"uuid\":\"bbe80fa3-b8e3-44c5-9574-5758a55378fd\"},{\"content\":{\"side\":\"TOP\"},\"type\":\"ConnectorPlacement.EquallySpacedRectSide\",\"uuid\":\"410005e2-e10b-4d3e-a617-d51b1ea5de7e\"}]},\"type\":\"ConnectorPlacement.EquallySpacedConnector\",\"uuid\":\"b66a347a-e5b4-46b1-8a3f-28cf70f30a27\"}],\"packageUris\":[\"http://schema.mathworks.com/mf0/Connector/R2020b\"],\"version\":\"1.0\"}"
  Feed controller : Subsystem
      settings: PortSchema="{\"entries\":[{\"content\":{\"headerSize\":26,\"margin\":15,\"minimumSpacing\":25,\"sides\":[{\"content\":{\"connectorIds\":[\"In1\",\"LConn1\"]},\"type\":\"ConnectorPlacement.EquallySpacedRectSide\",\"uuid\":\"fbe4f8e6-132c-4a0c-8c4c-52d0209da778\"},{\"content\":{\"connectorIds\":[\"Out1\",\"Out2\"],\"side\":\"RIGHT\"},\"type\":\"ConnectorPlacement.EquallySpacedRectSide\",\"uuid\":\"bbe80fa3-b8e3-44c5-9574-5758a55378fd\"},{\"content\":{\"side\":\"TOP\"},\"type\":\"ConnectorPlacement.EquallySpacedRectSide\",\"uuid\":\"410005e2-e10b-4d3e-a617-d51b1ea5de7e\"}]},\"type\":\"ConnectorPlacement.EquallySpacedConnector\",\"uuid\":\"b66a347a-e5b4-46b1-8a3f-28cf70f30a27\"}],\"packageUris\":[\"http://schema.mathworks.com/mf0/Connector/R2020b\"],\"version\":\"1.0\"}"
  Header tank switchover valve : Subsystem
      settings: PortSchema="{\"entries\":[{\"content\":{\"headerSize\":26,\"margin\":15,\"minimumSpacing\":25,\"sides\":[{\"content\":{\"connectorIds\":[\"LConn1\",\"LConn2\",\"In1\",\"LConn3\"]},\"type\":\"ConnectorPlacement.EquallySpacedRectSide\",\"uuid\":\"fbe4f8e6-132c-4a0c-8c4c-52d0209da778\"},{\"content\":{\"connectorIds\":[\"RConn1\"],\"side\":\"RIGHT\"},\"type\":\"ConnectorPlacement.EquallySpacedRectSide\",\"uuid\":\"bbe80fa3-b8e3-44c5-9574-5758a55378fd\"},{\"content\":{\"side\":\"TOP\"},\"type\":\"ConnectorPlacement.EquallySpacedRectSide\",\"uuid\":\"410005e2-e10b-4d3e-a617-d51b1ea5de7e\"}]},\"type\":\"ConnectorPlacement.EquallySpacedConnector\",\"uuid\":\"b66a347a-e5b4-46b1-8a3f-28cf70f30a27\"}],\"packageUris\":[\"http://schema.mathworks.com/mf0/Connector/R2020b\"],\"version\":\"1.0\"}"
  Main tank outlet valve (prevalve) : Subsystem
      settings: PortSchema="{\"entries\":[{\"content\":{\"headerSize\":26,\"margin\":15,\"minimumSpacing\":25,\"sides\":[{\"content\":{\"connectorIds\":[\"LConn1\",\"LConn2\",\"LConn3\",\"In1\"]},\"type\":\"ConnectorPlacement.EquallySpacedRectSide\",\"uuid\":\"fbe4f8e6-132c-4a0c-8c4c-52d0209da778\"},{\"content\":{\"connectorIds\":[\"RConn1\"],\"side\":\"RIGHT\"},\"type\":\"ConnectorPlacement.EquallySpacedRectSide\",\"uuid\":\"bbe80fa3-b8e3-44c5-9574-5758a55378fd\"},{\"content\":{\"side\":\"TOP\"},\"type\":\"ConnectorPlacement.EquallySpacedRectSide\",\"uuid\":\"410005e2-e10b-4d3e-a617-d51b1ea5de7e\"}]},\"type\":\"ConnectorPlacement.EquallySpacedConnector\",\"uuid\":\"b66a347a-e5b4-46b1-8a3f-28cf70f30a27\"}],\"packageUris\":[\"http://schema.mathworks.com/mf0/Connector/R2020b\"],\"version\":\"1.0\"}"
  IF-SDM-STP-01 : PMIOPort  Side=Right  ConnectionType=Bus: LiquidPropellantFeed
  IF-SNG-SPV-01 : PMIOPort  Port=2  Side=Left  ConnectionType=Bus: PneumaticActuationGas
  IF-SOT-SPV-01 : PMIOPort  Port=3  Side=Left  ConnectionType=Bus: LiquidPropellantFeed
  IF-SFT-SPV-01 : PMIOPort  Port=4  Side=Left  ConnectionType=Bus: LiquidPropellantFeed
  IF-SLT-SHV-01 : PMIOPort  Port=5  Side=Left  ConnectionType=Bus: LiquidPropellantFeed
  IF-SCH-SHV-01 : PMIOPort  Port=6  Side=Left  ConnectionType=Bus: LiquidPropellantFeed
  IF-SNG-SHV-01 : PMIOPort  Port=7  Side=Left  ConnectionType=Bus: PneumaticActuationGas
  IF-PWR-SFC-01 : PMIOPort  Port=8  Side=Left  ConnectionType=Bus: ElectricalPower
  wires:
  Feed controller/2(IF-SFC-SHV-01) -> Header tank switchover valve/1(IF-SFC-SHV-01)
  Bus Element In1/1 -> Feed controller/1(IF-GNC-SFC-01)
  Feed controller/1(IF-SFC-SPV-01) -> Main tank outlet valve (prevalve)/1(IF-SFC-SPV-01)
  connections:
  Header tank switchover valve/RConn1 -- Distribution manifold/LConn1
  IF-SFT-SPV-01/RConn1 -- Main tank outlet valve (prevalve)/LConn3
  IF-SLT-SHV-01/RConn1 -- Header tank switchover valve/LConn1
  IF-SCH-SHV-01/RConn1 -- Header tank switchover valve/LConn2
  IF-SNG-SHV-01/RConn1 -- Header tank switchover valve/LConn3
  IF-SNG-SPV-01/RConn1 -- Main tank outlet valve (prevalve)/LConn1
  Main tank outlet valve (prevalve)/RConn1 -- Distribution manifold/LConn2
  IF-SOT-SPV-01/RConn1 -- Main tank outlet valve (prevalve)/LConn2
  Distribution manifold/RConn1 -- IF-SDM-STP-01/RConn1
  IF-PWR-SFC-01/RConn1 -- Feed controller/LConn1

== system StarshipSystemModel/Starship/Propellent system/Ship propellant System/Ground propellant interface ==
  CH4 quick-disconnect panel : Subsystem
      settings: PortSchema="{\"entries\":[{\"content\":{\"headerSize\":26,\"margin\":15,\"minimumSpacing\":25,\"sides\":[{\"content\":{\"connectorIds\":[\"LConn1\"]},\"type\":\"ConnectorPlacement.EquallySpacedRectSide\",\"uuid\":\"fbe4f8e6-132c-4a0c-8c4c-52d0209da778\"},{\"content\":{\"connectorIds\":[\"RConn1\"],\"side\":\"RIGHT\"},\"type\":\"ConnectorPlacement.EquallySpacedRectSide\",\"uuid\":\"bbe80fa3-b8e3-44c5-9574-5758a55378fd\"},{\"content\":{\"side\":\"TOP\"},\"type\":\"ConnectorPlacement.EquallySpacedRectSide\",\"uuid\":\"410005e2-e10b-4d3e-a617-d51b1ea5de7e\"}]},\"type\":\"ConnectorPlacement.EquallySpacedConnector\",\"uuid\":\"b66a347a-e5b4-46b1-8a3f-28cf70f30a27\"}],\"packageUris\":[\"http://schema.mathworks.com/mf0/Connector/R2020b\"],\"version\":\"1.0\"}"
  LOX quick-disconnect panel : Subsystem
      settings: PortSchema="{\"entries\":[{\"content\":{\"headerSize\":26,\"margin\":15,\"minimumSpacing\":25,\"sides\":[{\"content\":{\"connectorIds\":[\"LConn1\"]},\"type\":\"ConnectorPlacement.EquallySpacedRectSide\",\"uuid\":\"fbe4f8e6-132c-4a0c-8c4c-52d0209da778\"},{\"content\":{\"connectorIds\":[\"RConn1\"],\"side\":\"RIGHT\"},\"type\":\"ConnectorPlacement.EquallySpacedRectSide\",\"uuid\":\"bbe80fa3-b8e3-44c5-9574-5758a55378fd\"},{\"content\":{\"side\":\"TOP\"},\"type\":\"ConnectorPlacement.EquallySpacedRectSide\",\"uuid\":\"410005e2-e10b-4d3e-a617-d51b1ea5de7e\"}]},\"type\":\"ConnectorPlacement.EquallySpacedConnector\",\"uuid\":\"b66a347a-e5b4-46b1-8a3f-28cf70f30a27\"}],\"packageUris\":[\"http://schema.mathworks.com/mf0/Connector/R2020b\"],\"version\":\"1.0\"}"
  Purge/pressurant ground QD : Subsystem
      settings: PortSchema="{\"entries\":[{\"content\":{\"headerSize\":26,\"margin\":15,\"minimumSpacing\":25,\"sides\":[{\"content\":{\"connectorIds\":[\"LConn1\"]},\"type\":\"ConnectorPlacement.EquallySpacedRectSide\",\"uuid\":\"fbe4f8e6-132c-4a0c-8c4c-52d0209da778\"},{\"content\":{\"connectorIds\":[\"RConn1\",\"RConn2\",\"RConn3\"],\"side\":\"RIGHT\"},\"type\":\"ConnectorPlacement.EquallySpacedRectSide\",\"uuid\":\"bbe80fa3-b8e3-44c5-9574-5758a55378fd\"},{\"content\":{\"side\":\"TOP\"},\"type\":\"ConnectorPlacement.EquallySpacedRectSide\",\"uuid\":\"410005e2-e10b-4d3e-a617-d51b1ea5de7e\"}]},\"type\":\"ConnectorPlacement.EquallySpacedConnector\",\"uuid\":\"b66a347a-e5b4-46b1-8a3f-28cf70f30a27\"}],\"packageUris\":[\"http://schema.mathworks.com/mf0/Connector/R2020b\"],\"version\":\"1.0\"}"
  IF-GND-SLQ-01 : PMIOPort  Side=Left
  IF-GND-SCQ-01 : PMIOPort  Port=2  Side=Left
  IF-GND-SPQ-01 : PMIOPort  Port=3  Side=Left  ConnectionType=Bus: GroundPressurantSupply
  IF-SCQ-SFT-01 : PMIOPort  Port=4  Side=Right  ConnectionType=Bus: LiquidPropellantFeed
  IF-SPQ-SSG-01 : PMIOPort  Port=5  Side=Right  ConnectionType=Bus: GroundPressurantSupply
  IF-SPQ-SNG-01 : PMIOPort  Port=6  Side=Right  ConnectionType=Bus: GroundPressurantSupply
  IF-SPQ-SPR-01 : PMIOPort  Port=7  Side=Right  ConnectionType=Bus: GroundPressurantSupply
  IF-SLQ-SOT-01 : PMIOPort  Port=8  Side=Right  ConnectionType=Bus: LiquidPropellantFeed
  connections:
  Purge/pressurant ground QD/RConn3 -- IF-SPQ-SNG-01/RConn1
  Purge/pressurant ground QD/RConn1 -- IF-SPQ-SSG-01/RConn1
  IF-GND-SLQ-01/RConn1 -- LOX quick-disconnect panel/LConn1
  IF-GND-SCQ-01/RConn1 -- CH4 quick-disconnect panel/LConn1
  IF-GND-SPQ-01/RConn1 -- Purge/pressurant ground QD/LConn1
  LOX quick-disconnect panel/RConn1 -- IF-SLQ-SOT-01/RConn1
  Purge/pressurant ground QD/RConn2 -- IF-SPQ-SPR-01/RConn1
  CH4 quick-disconnect panel/RConn1 -- IF-SCQ-SFT-01/RConn1

== system StarshipSystemModel/Starship/Propellent system/Ship propellant System/Pressurization, purge & venting ==
  Bus Element In1 : Inport  PortName=IF-GNC-SPR-01
  Autogenous pressurization regulator : Subsystem
      settings: PortSchema="{\"entries\":[{\"content\":{\"headerSize\":26,\"margin\":15,\"minimumSpacing\":25,\"sides\":[{\"content\":{\"connectorIds\":[\"LConn1\",\"LConn2\",\"In1\",\"LConn3\"]},\"type\":\"ConnectorPlacement.EquallySpacedRectSide\",\"uuid\":\"fbe4f8e6-132c-4a0c-8c4c-52d0209da778\"},{\"content\":{\"connectorIds\":[\"RConn1\",\"Out1\",\"Out2\",\"RConn2\",\"RConn3\",\"Out3\"],\"side\":\"RIGHT\"},\"type\":\"ConnectorPlacement.EquallySpacedRectSide\",\"uuid\":\"bbe80fa3-b8e3-44c5-9574-5758a55378fd\"},{\"content\":{\"side\":\"TOP\"},\"type\":\"ConnectorPlacement.EquallySpacedRectSide\",\"uuid\":\"410005e2-e10b-4d3e-a617-d51b1ea5de7e\"}]},\"type\":\"ConnectorPlacement.EquallySpacedConnector\",\"uuid\":\"b66a347a-e5b4-46b1-8a3f-28cf70f30a27\"}],\"packageUris\":[\"http://schema.mathworks.com/mf0/Connector/R2020b\"],\"version\":\"1.0\"}"
  Pneumatic actuation gas COPVs : Subsystem
      settings: PortSchema="{\"entries\":[{\"content\":{\"headerSize\":26,\"margin\":15,\"minimumSpacing\":25,\"sides\":[{\"content\":{\"connectorIds\":[\"LConn1\"]},\"type\":\"ConnectorPlacement.EquallySpacedRectSide\",\"uuid\":\"fbe4f8e6-132c-4a0c-8c4c-52d0209da778\"},{\"content\":{\"connectorIds\":[\"RConn1\",\"RConn2\",\"RConn3\",\"RConn4\"],\"side\":\"RIGHT\"},\"type\":\"ConnectorPlacement.EquallySpacedRectSide\",\"uuid\":\"bbe80fa3-b8e3-44c5-9574-5758a55378fd\"},{\"content\":{\"side\":\"TOP\"},\"type\":\"ConnectorPlacement.EquallySpacedRectSide\",\"uuid\":\"410005e2-e10b-4d3e-a617-d51b1ea5de7e\"}]},\"type\":\"ConnectorPlacement.EquallySpacedConnector\",\"uuid\":\"b66a347a-e5b4-46b1-8a3f-28cf70f30a27\"}],\"packageUris\":[\"http://schema.mathworks.com/mf0/Connector/R2020b\"],\"version\":\"1.0\"}"
  Spin-start & igniter gas COPVs : Subsystem
      settings: PortSchema="{\"entries\":[{\"content\":{\"headerSize\":26,\"margin\":15,\"minimumSpacing\":25,\"sides\":[{\"content\":{\"connectorIds\":[\"LConn1\"]},\"type\":\"ConnectorPlacement.EquallySpacedRectSide\",\"uuid\":\"fbe4f8e6-132c-4a0c-8c4c-52d0209da778\"},{\"content\":{\"connectorIds\":[\"RConn1\"],\"side\":\"RIGHT\"},\"type\":\"ConnectorPlacement.EquallySpacedRectSide\",\"uuid\":\"bbe80fa3-b8e3-44c5-9574-5758a55378fd\"},{\"content\":{\"side\":\"TOP\"},\"type\":\"ConnectorPlacement.EquallySpacedRectSide\",\"uuid\":\"410005e2-e10b-4d3e-a617-d51b1ea5de7e\"}]},\"type\":\"ConnectorPlacement.EquallySpacedConnector\",\"uuid\":\"b66a347a-e5b4-46b1-8a3f-28cf70f30a27\"}],\"packageUris\":[\"http://schema.mathworks.com/mf0/Connector/R2020b\"],\"version\":\"1.0\"}"
  Vent & relief valves : Subsystem
      settings: PortSchema="{\"entries\":[{\"content\":{\"headerSize\":26,\"margin\":15,\"minimumSpacing\":25,\"sides\":[{\"content\":{\"connectorIds\":[\"In1\",\"LConn1\",\"LConn2\",\"LConn3\"]},\"type\":\"ConnectorPlacement.EquallySpacedRectSide\",\"uuid\":\"fbe4f8e6-132c-4a0c-8c4c-52d0209da778\"},{\"content\":{\"side\":\"RIGHT\"},\"type\":\"ConnectorPlacement.EquallySpacedRectSide\",\"uuid\":\"bbe80fa3-b8e3-44c5-9574-5758a55378fd\"},{\"content\":{\"side\":\"TOP\"},\"type\":\"ConnectorPlacement.EquallySpacedRectSide\",\"uuid\":\"410005e2-e10b-4d3e-a617-d51b1ea5de7e\"}]},\"type\":\"ConnectorPlacement.EquallySpacedConnector\",\"uuid\":\"b66a347a-e5b4-46b1-8a3f-28cf70f30a27\"}],\"packageUris\":[\"http://schema.mathworks.com/mf0/Connector/R2020b\"],\"version\":\"1.0\"}"
  IF-SSG-SIG-01 : PMIOPort  Side=Right  ConnectionType=Bus: SpinStartIgniterGas
  IF-SPR-SOT-01 : PMIOPort  Port=2  Side=Right  ConnectionType=Bus: AutogenousPressurantGas
  IF-SPR-SFT-01 : PMIOPort  Port=3  Side=Right  ConnectionType=Bus: AutogenousPressurantGas
  IF-SNG-SPV-01 : PMIOPort  Port=4  Side=Right  ConnectionType=Bus: PneumaticActuationGas
  IF-SNG-SHV-01 : PMIOPort  Port=5  Side=Right  ConnectionType=Bus: PneumaticActuationGas
  IF-SNG-SVC-01 : PMIOPort  Port=6  Side=Right  ConnectionType=Bus: PneumaticActuationGas
  IF-SPR-RVM-01 : PMIOPort  Port=7  Side=Right  ConnectionType=Bus: CombustionGasFeed
  IF-STP-SPR-01 : PMIOPort  Port=8  Side=Left  ConnectionType=Bus: AutogenousPressurantGas
  IF-SOT-SVV-01 : PMIOPort  Port=9  Side=Left
  IF-SFT-SVV-01 : PMIOPort  Port=10  Side=Left
  IF-SPQ-SSG-01 : PMIOPort  Port=11  Side=Left  ConnectionType=Bus: GroundPressurantSupply
  IF-SPQ-SNG-01 : PMIOPort  Port=12  Side=Left  ConnectionType=Bus: GroundPressurantSupply
  IF-SPQ-SPR-01 : PMIOPort  Port=13  Side=Left  ConnectionType=Bus: GroundPressurantSupply
  IF-PWR-SPR-01 : PMIOPort  Port=14  Side=Left  ConnectionType=Bus: ElectricalPower
  Bus Element Out1 : Outport  PortName=IF-SPR-SAF-01
  Bus Element Out2 : Outport  Port=2  PortName=IF-SPR-STA-01
  wires:
  Autogenous pressurization regulator/1(IF-SPR-SAF-01) -> Bus Element Out1/1
  Bus Element In1/1 -> Autogenous pressurization regulator/1(IF-GNC-SPR-01)
  Autogenous pressurization regulator/2(IF-SPR-STA-01) -> Bus Element Out2/1
  Autogenous pressurization regulator/3(IF-SPR-SVV-01) -> Vent & relief valves/1(IF-SPR-SVV-01)
  connections:
  IF-SPQ-SSG-01/RConn1 -- Spin-start & igniter gas COPVs/LConn1
  IF-STP-SPR-01/RConn1 -- Autogenous pressurization regulator/LConn1
  IF-SPQ-SNG-01/RConn1 -- Pneumatic actuation gas COPVs/LConn1
  IF-SOT-SVV-01/RConn1 -- Vent & relief valves/LConn1
  IF-SPQ-SPR-01/RConn1 -- Autogenous pressurization regulator/LConn2
  Autogenous pressurization regulator/RConn1 -- IF-SPR-RVM-01/RConn1
  Pneumatic actuation gas COPVs/RConn1 -- IF-SNG-SPV-01/RConn1
  Autogenous pressurization regulator/RConn2 -- IF-SPR-SOT-01/RConn1
  Pneumatic actuation gas COPVs/RConn2 -- IF-SNG-SHV-01/RConn1
  Autogenous pressurization regulator/RConn3 -- IF-SPR-SFT-01/RConn1
  IF-SFT-SVV-01/RConn1 -- Vent & relief valves/LConn2
  Pneumatic actuation gas COPVs/RConn3 -- IF-SNG-SVC-01/RConn1
  Pneumatic actuation gas COPVs/RConn4 -- Vent & relief valves/LConn3
  Spin-start & igniter gas COPVs/RConn1 -- IF-SSG-SIG-01/RConn1
  IF-PWR-SPR-01/RConn1 -- Autogenous pressurization regulator/LConn3

== system StarshipSystemModel/Starship/Propellent system/Ship propellant System/Ship propellant tanks ==
  Anti-slosh baffles : Subsystem
      settings: PortSchema="{\"entries\":[{\"content\":{\"headerSize\":26,\"margin\":15,\"minimumSpacing\":25,\"sides\":[{\"content\":{},\"type\":\"ConnectorPlacement.EquallySpacedRectSide\",\"uuid\":\"fbe4f8e6-132c-4a0c-8c4c-52d0209da778\"},{\"content\":{\"side\":\"RIGHT\"},\"type\":\"ConnectorPlacement.EquallySpacedRectSide\",\"uuid\":\"bbe80fa3-b8e3-44c5-9574-5758a55378fd\"},{\"content\":{\"side\":\"TOP\"},\"type\":\"ConnectorPlacement.EquallySpacedRectSide\",\"uuid\":\"410005e2-e10b-4d3e-a617-d51b1ea5de7e\"}]},\"type\":\"ConnectorPlacement.EquallySpacedConnector\",\"uuid\":\"b66a347a-e5b4-46b1-8a3f-28cf70f30a27\"}],\"packageUris\":[\"http://schema.mathworks.com/mf0/Connector/R2020b\"],\"version\":\"1.0\"}"
  CH4 header tank : Subsystem
      settings: PortSchema="{\"entries\":[{\"content\":{\"headerSize\":26,\"margin\":15,\"minimumSpacing\":25,\"sides\":[{\"content\":{},\"type\":\"ConnectorPlacement.EquallySpacedRectSide\",\"uuid\":\"fbe4f8e6-132c-4a0c-8c4c-52d0209da778\"},{\"content\":{\"connectorIds\":[\"RConn1\"],\"side\":\"RIGHT\"},\"type\":\"ConnectorPlacement.EquallySpacedRectSide\",\"uuid\":\"bbe80fa3-b8e3-44c5-9574-5758a55378fd\"},{\"content\":{\"side\":\"TOP\"},\"type\":\"ConnectorPlacement.EquallySpacedRectSide\",\"uuid\":\"410005e2-e10b-4d3e-a617-d51b1ea5de7e\"}]},\"type\":\"ConnectorPlacement.EquallySpacedConnector\",\"uuid\":\"b66a347a-e5b4-46b1-8a3f-28cf70f30a27\"}],\"packageUris\":[\"http://schema.mathworks.com/mf0/Connector/R2020b\"],\"version\":\"1.0\"}"
  CH4 main tank : Subsystem
      settings: PortSchema="{\"entries\":[{\"content\":{\"headerSize\":26,\"margin\":15,\"minimumSpacing\":25,\"sides\":[{\"content\":{\"connectorIds\":[\"LConn1\",\"LConn2\"]},\"type\":\"ConnectorPlacement.EquallySpacedRectSide\",\"uuid\":\"fbe4f8e6-132c-4a0c-8c4c-52d0209da778\"},{\"content\":{\"connectorIds\":[\"RConn1\",\"RConn2\"],\"side\":\"RIGHT\"},\"type\":\"ConnectorPlacement.EquallySpacedRectSide\",\"uuid\":\"bbe80fa3-b8e3-44c5-9574-5758a55378fd\"},{\"content\":{\"side\":\"TOP\"},\"type\":\"ConnectorPlacement.EquallySpacedRectSide\",\"uuid\":\"410005e2-e10b-4d3e-a617-d51b1ea5de7e\"}]},\"type\":\"ConnectorPlacement.EquallySpacedConnector\",\"uuid\":\"b66a347a-e5b4-46b1-8a3f-28cf70f30a27\"}],\"packageUris\":[\"http://schema.mathworks.com/mf0/Connector/R2020b\"],\"version\":\"1.0\"}"
  CH4 transfer tube (downcomer) : Subsystem
      settings: PortSchema="{\"entries\":[{\"content\":{\"headerSize\":26,\"margin\":15,\"minimumSpacing\":25,\"sides\":[{\"content\":{},\"type\":\"ConnectorPlacement.EquallySpacedRectSide\",\"uuid\":\"fbe4f8e6-132c-4a0c-8c4c-52d0209da778\"},{\"content\":{\"side\":\"RIGHT\"},\"type\":\"ConnectorPlacement.EquallySpacedRectSide\",\"uuid\":\"bbe80fa3-b8e3-44c5-9574-5758a55378fd\"},{\"content\":{\"side\":\"TOP\"},\"type\":\"ConnectorPlacement.EquallySpacedRectSide\",\"uuid\":\"410005e2-e10b-4d3e-a617-d51b1ea5de7e\"}]},\"type\":\"ConnectorPlacement.EquallySpacedConnector\",\"uuid\":\"b66a347a-e5b4-46b1-8a3f-28cf70f30a27\"}],\"packageUris\":[\"http://schema.mathworks.com/mf0/Connector/R2020b\"],\"version\":\"1.0\"}"
  Common dome : Subsystem
      settings: PortSchema="{\"entries\":[{\"content\":{\"headerSize\":26,\"margin\":15,\"minimumSpacing\":25,\"sides\":[{\"content\":{},\"type\":\"ConnectorPlacement.EquallySpacedRectSide\",\"uuid\":\"fbe4f8e6-132c-4a0c-8c4c-52d0209da778\"},{\"content\":{\"side\":\"RIGHT\"},\"type\":\"ConnectorPlacement.EquallySpacedRectSide\",\"uuid\":\"bbe80fa3-b8e3-44c5-9574-5758a55378fd\"},{\"content\":{\"side\":\"TOP\"},\"type\":\"ConnectorPlacement.EquallySpacedRectSide\",\"uuid\":\"410005e2-e10b-4d3e-a617-d51b1ea5de7e\"}]},\"type\":\"ConnectorPlacement.EquallySpacedConnector\",\"uuid\":\"b66a347a-e5b4-46b1-8a3f-28cf70f30a27\"}],\"packageUris\":[\"http://schema.mathworks.com/mf0/Connector/R2020b\"],\"version\":\"1.0\"}"
  LOX header tank : Subsystem
      settings: PortSchema="{\"entries\":[{\"content\":{\"headerSize\":26,\"margin\":15,\"minimumSpacing\":25,\"sides\":[{\"content\":{},\"type\":\"ConnectorPlacement.EquallySpacedRectSide\",\"uuid\":\"fbe4f8e6-132c-4a0c-8c4c-52d0209da778\"},{\"content\":{\"connectorIds\":[\"RConn1\"],\"side\":\"RIGHT\"},\"type\":\"ConnectorPlacement.EquallySpacedRectSide\",\"uuid\":\"bbe80fa3-b8e3-44c5-9574-5758a55378fd\"},{\"content\":{\"side\":\"TOP\"},\"type\":\"ConnectorPlacement.EquallySpacedRectSide\",\"uuid\":\"410005e2-e10b-4d3e-a617-d51b1ea5de7e\"}]},\"type\":\"ConnectorPlacement.EquallySpacedConnector\",\"uuid\":\"b66a347a-e5b4-46b1-8a3f-28cf70f30a27\"}],\"packageUris\":[\"http://schema.mathworks.com/mf0/Connector/R2020b\"],\"version\":\"1.0\"}"
  LOX main tank : Subsystem
      settings: PortSchema="{\"entries\":[{\"content\":{\"headerSize\":26,\"margin\":15,\"minimumSpacing\":25,\"sides\":[{\"content\":{\"connectorIds\":[\"LConn2\",\"LConn3\"]},\"type\":\"ConnectorPlacement.EquallySpacedRectSide\",\"uuid\":\"fbe4f8e6-132c-4a0c-8c4c-52d0209da778\"},{\"content\":{\"connectorIds\":[\"LConn1\",\"RConn1\",\"RConn2\"],\"side\":\"RIGHT\"},\"type\":\"ConnectorPlacement.EquallySpacedRectSide\",\"uuid\":\"bbe80fa3-b8e3-44c5-9574-5758a55378fd\"},{\"content\":{\"side\":\"TOP\"},\"type\":\"ConnectorPlacement.EquallySpacedRectSide\",\"uuid\":\"410005e2-e10b-4d3e-a617-d51b1ea5de7e\"}]},\"type\":\"ConnectorPlacement.EquallySpacedConnector\",\"uuid\":\"b66a347a-e5b4-46b1-8a3f-28cf70f30a27\"}],\"packageUris\":[\"http://schema.mathworks.com/mf0/Connector/R2020b\"],\"version\":\"1.0\"}"
  IF-SOT-SPV-01 : PMIOPort  Side=Right  ConnectionType=Bus: LiquidPropellantFeed
  IF-SFT-SPV-01 : PMIOPort  Port=2  Side=Right  ConnectionType=Bus: LiquidPropellantFeed
  IF-SFT-SVV-01 : PMIOPort  Port=3  Side=Right
  IF-SOT-SVV-01 : PMIOPort  Port=4  Side=Right
  IF-SLT-SHV-01 : PMIOPort  Port=5  Side=Right  ConnectionType=Bus: LiquidPropellantFeed
  IF-SCH-SHV-01 : PMIOPort  Port=6  Side=Right  ConnectionType=Bus: LiquidPropellantFeed
  IF-SOT-PRS-01 : PMIOPort  Port=7  Side=Left  ConnectionType=Bus: StructuralLoad
  IF-SPR-SFT-01 : PMIOPort  Port=8  Side=Left  ConnectionType=Bus: AutogenousPressurantGas
  IF-SPR-SOT-01 : PMIOPort  Port=9  Side=Left  ConnectionType=Bus: AutogenousPressurantGas
  IF-SLQ-SOT-01 : PMIOPort  Port=10  Side=Left  ConnectionType=Bus: LiquidPropellantFeed
  IF-SCQ-SFT-01 : PMIOPort  Port=11  Side=Left  ConnectionType=Bus: LiquidPropellantFeed
  connections:
  CH4 header tank/RConn1 -- IF-SCH-SHV-01/RConn1
  LOX header tank/RConn1 -- IF-SLT-SHV-01/RConn1
  IF-SPR-SOT-01/RConn1 -- LOX main tank/LConn2
  IF-SPR-SFT-01/RConn1 -- CH4 main tank/LConn1
  IF-SLQ-SOT-01/RConn1 -- LOX main tank/LConn3
  IF-SCQ-SFT-01/RConn1 -- CH4 main tank/LConn2
  LOX main tank/RConn1 -- IF-SOT-SPV-01/RConn1
  CH4 main tank/RConn2 -- IF-SFT-SVV-01/RConn1
  LOX main tank/RConn2 -- IF-SOT-SVV-01/RConn1
  CH4 main tank/RConn1 -- IF-SFT-SPV-01/RConn1
  IF-SOT-PRS-01/RConn1 -- LOX main tank/LConn1

== system StarshipSystemModel/Starship/Propulsion/Booster main engines/Combustion Chamber  ==
  IF-BPB-BCC-01 : PMIOPort  Side=Left  ConnectionType=Bus: CombustionGasFeed
  IF-BCC-BNZ-01 : PMIOPort  Port=2  Side=Right  ConnectionType=Bus: CombustionGasFeed
